simulink model "Simulacion_Trifasico_PID_v8"  (R2024a)
settings: Solver=ode3  StartTime=0  StopTime=tend  FixedStep=0.01  RelTol=1e-3
values from neighbouring files (symbols this model uses):
  ts = 0.1    [Fuzzy_init.m]    (also in MPC_linealizar_v6.m)
libraries: simulink x6, eeStairGenerator x6
settings Model: Creator=Ivan  LastModifiedBy=Ivan
settings DebuggingCC: UnderSpecifiedDimensionMsg=warning
settings ConfigComp: PLC_TargetIDE=tiaportal  PLC_MultiTBSigbuilderTimeRange=off  PLC_FoldFBCallOutputVar=off  PLC_RemoveUnusedSSMethodCallArguments=off  PLC_UseCallOutputArgSyntax=off  PLC_EnableUnsignedAndDoubleTypes=off  PLC_EnableUDTSplitting=off  PLC_MaxFieldsInUDT=500  PLC_InlineEnumCastFunction=off

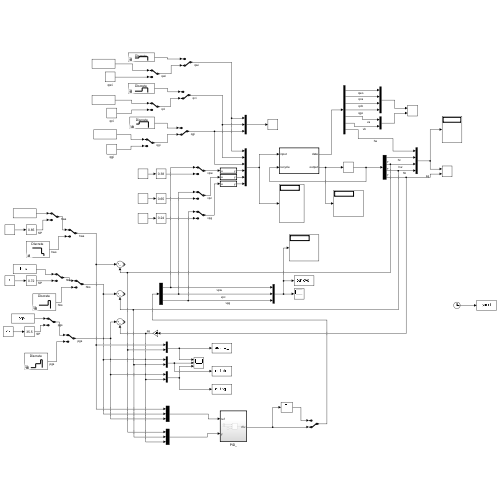
[thumbnail: Simulink's stored preview of the top-level diagram]
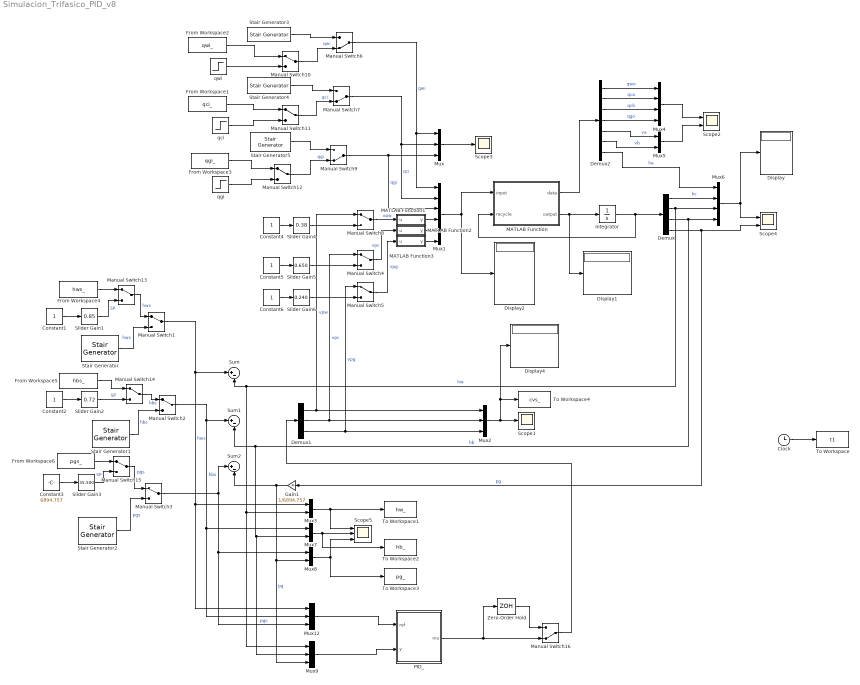
== system Simulacion_Trifasico_PID_v8 ==
  Clock : Clock
  Constant{1..2,4..6} (5 alike) : Constant
  Constant3 : Constant  Value=6894.757
  Demux : Demux
  Demux1 : Demux  Outputs=3
  Demux2 : Demux  Outputs=7
  Display{,1..2,4} (4 alike) : Display
  From Workspace1 : FromWorkspace  VariableName=qci_  SampleTime=ts
  From Workspace2 : FromWorkspace  VariableName=qwi_  SampleTime=ts
  From Workspace3 : FromWorkspace  VariableName=qgi_  SampleTime=ts
  From Workspace4 : FromWorkspace  VariableName=hws_  SampleTime=ts
  From Workspace5 : FromWorkspace  VariableName=hbs_  SampleTime=ts
  From Workspace6 : FromWorkspace  VariableName=pgs_  SampleTime=ts
  Gain1 : Gain  Gain=1/6894.757
  Integrator : Integrator  InitialCondition=[0.4737; 0.80; 0.72; 37*6894.757]  LimitOutput=on  LowerSaturationLimit=0
  MATLAB Function : MATLAB Function  TreatAsAtomicUnit=on
  MATLAB Function1 : MATLAB Function  TreatAsAtomicUnit=on
  MATLAB Function2 : MATLAB Function  TreatAsAtomicUnit=on
  MATLAB Function3 : MATLAB Function  TreatAsAtomicUnit=on
  Manual Switch{1..5,8,10..15} (12 alike) : ManualSwitch
  Manual Switch{6..7,9,16} (4 alike) : ManualSwitch  CurrentSetting=0
  Mux{,2,9,12} (4 alike) : Mux  Inputs=3
  Mux1 : Mux  Inputs=6
  Mux{3,5,7..8} (4 alike) : Mux  Inputs=2
  Mux4 : Mux
  Mux6 : Mux
  PID_ : Subsystem  TreatAsAtomicUnit=on  SystemSampleTime=0.1
  Scope1 : Scope
  Scope2 : Scope  NumInputPorts=2
  Scope3 : Scope
  Scope4 : Scope  NumInputPorts=2
  Scope5 : Scope  NumInputPorts=3
  Slider Gain1 : simulink/Math Operations/Slider Gain  gain=0.85  low=0  high=1
  Slider Gain2 : simulink/Math Operations/Slider Gain  gain=0.72  low=0  high=1
  Slider Gain3 : simulink/Math Operations/Slider Gain  gain=35.500  low=0  high=50
  Slider Gain4 : simulink/Math Operations/Slider Gain  gain=0.38  low=0  high=1
  Slider Gain5 : simulink/Math Operations/Slider Gain  gain=0.650  low=0  high=1
  Slider Gain6 : simulink/Math Operations/Slider Gain  gain=0.240  low=0  high=1
  Stair Generator : eeStairGenerator/Stair Generator  LabelModeActiveChoice=Discrete  TimeInput=[0 2000 2500]  AmplitudeInput=[0.85 0.80 0.78]  SampleTime=0.01  RepeatPattern=off  OutDataTypeStr=double
      settings: LibrarySourceBlock=ee_sl_lib/General Control/Stair Generator
  Stair Generator1 : eeStairGenerator/Stair Generator  LabelModeActiveChoice=Discrete  TimeInput=[0 2250 2750]  AmplitudeInput=[0.72 0.75 0.70]  SampleTime=0.01  RepeatPattern=off  OutDataTypeStr=double
      settings: LibrarySourceBlock=ee_sl_lib/General Control/Stair Generator
  Stair Generator2 : eeStairGenerator/Stair Generator  LabelModeActiveChoice=Discrete  TimeInput="[0 1500 3000  3500]"  AmplitudeInput=[35 40 45 35]  SampleTime=0.01  RepeatPattern=off  OutDataTypeStr=double
      settings: LibrarySourceBlock=ee_sl_lib/General Control/Stair Generator
  Stair Generator3 : eeStairGenerator/Stair Generator  LabelModeActiveChoice=Discrete  TimeInput=[0 1000 3250]  AmplitudeInput=[0.1374 0.1774 0.0474]  SampleTime=0.01  RepeatPattern=off  OutDataTypeStr=double
      settings: LibrarySourceBlock=ee_sl_lib/General Control/Stair Generator
  Stair Generator4 : eeStairGenerator/Stair Generator  LabelModeActiveChoice=Discrete  TimeInput=[0 1750 3100]  AmplitudeInput=[0.0711 0.1815 0.0298]  SampleTime=0.01  RepeatPattern=off  OutDataTypeStr=double
      settings: LibrarySourceBlock=ee_sl_lib/General Control/Stair Generator
  Stair Generator5 : eeStairGenerator/Stair Generator  LabelModeActiveChoice=Discrete  TimeInput=[0 1000 3750]  AmplitudeInput=[0.4906 0.79606 0.006]  SampleTime=0.01  RepeatPattern=off  OutDataTypeStr=double
      settings: LibrarySourceBlock=ee_sl_lib/General Control/Stair Generator
  Sum : Sum  Inputs=|+-
  Sum1 : Sum  Inputs=|+-
  Sum2 : Sum  Inputs=|+-
  To Workspace : ToWorkspace  VariableName=t1  SampleTime=0.1
  To Workspace1 : ToWorkspace  VariableName=hw_  SampleTime=0.1
  To Workspace2 : ToWorkspace  VariableName=hb_  SampleTime=0.1
  To Workspace3 : ToWorkspace  VariableName=pg_  SampleTime=0.1
  To Workspace4 : ToWorkspace  VariableName=cvs_  SampleTime=0.1
  Zero-Order Hold : ZeroOrderHold  SampleTime=-1
  qci : Step  After=.0711  SampleTime=0
  qgi : Step  After=.4906  SampleTime=0
  qwi : Step  After=.1374  SampleTime=0
  wires:
  Mux/1 -> Scope3/1
  Demux2/1 -> Mux4/1  "qwo"
  Demux2/2 -> Mux4/2  "qca"
  Demux2/3 -> Mux4/3  "qcb"
  Demux2/4 -> Mux4/4  "qgo"
  Demux2/5 -> Mux5/1  "va"
  Demux2/6 -> Mux5/2  "vb"
  Mux4/1 -> Scope2/1
  Mux5/1 -> Scope2/2
  Demux2/7 -> Mux6/1  "ha"
  Integrator/1 -> MATLAB Function/2(recycle), Demux/1
  Demux/1 -> Mux6/2  "hc"
  Demux/2 -> Mux9/1, Mux3/2, Sum/2, Mux6/3  "hw"
  Demux/3 -> Mux6/4, Sum1/2, Mux9/2, Mux7/2  "hb"
  Mux6/1 -> Display/1, Scope4/1
  Demux/4 -> Gain1/1, Scope4/2  "pg"
  Mux1/1 -> MATLAB Function/1(input), Display2/1
  MATLAB Function/2(output) -> Display1/1, Integrator/1
  MATLAB Function/1(data) -> Demux2/1
  Mux3/1 -> Scope5/1, To Workspace1/1
  Mux7/1 -> To Workspace2/1, Scope5/2
  Mux8/1 -> To Workspace3/1, Scope5/3
  Constant1/1 -> Slider Gain1/1
  Manual Switch1/1 -> Sum/1, Mux12/1, Mux3/1  "hws"
  Stair Generator/1 -> Manual Switch1/2  "hws"
  Constant2/1 -> Slider Gain2/1
  Manual Switch2/1 -> Sum1/1, Mux12/2, Mux7/1  "hbs"
  Constant3/1 -> Slider Gain3/1
  Manual Switch3/1 -> Sum2/1, Mux8/1, Mux12/3  "pgs"
  Stair Generator1/1 -> Manual Switch2/2  "hbs"
  Stair Generator2/1 -> Manual Switch3/2  "pgs"
  Constant4/1 -> Slider Gain4/1
  Slider Gain4/1 -> Manual Switch8/2
  Slider Gain5/1 -> Manual Switch4/2
  Constant5/1 -> Slider Gain5/1
  Slider Gain6/1 -> Manual Switch5/2
  Constant6/1 -> Slider Gain6/1
  Stair Generator3/1 -> Manual Switch6/1
  Stair Generator4/1 -> Manual Switch7/1
  Stair Generator5/1 -> Manual Switch9/1
  Manual Switch6/1 -> Mux1/1, Mux/1  "qwi"
  Manual Switch7/1 -> Mux/2, Mux1/2  "qci"
  Manual Switch9/1 -> Mux/3, Mux1/3  "qgi"
  Clock/1 -> To Workspace/1
  qwi/1 -> Manual Switch10/2
  Manual Switch10/1 -> Manual Switch6/2  "qwi"
  From Workspace2/1 -> Manual Switch10/1
  qci/1 -> Manual Switch11/2
  Manual Switch11/1 -> Manual Switch7/2  "qci"
  From Workspace1/1 -> Manual Switch11/1
  qgi/1 -> Manual Switch12/2
  Manual Switch12/1 -> Manual Switch9/2  "qgi"
  From Workspace3/1 -> Manual Switch12/1
  Slider Gain1/1 -> Manual Switch13/2  "SP"
  Manual Switch13/1 -> Manual Switch1/1  "hws"
  Slider Gain2/1 -> Manual Switch14/2  "SP"
  Manual Switch14/1 -> Manual Switch2/1  "hbs"
  Manual Switch15/1 -> Manual Switch3/1  "pgs"
  Slider Gain3/1 -> Manual Switch15/2  "SP"
  From Workspace4/1 -> Manual Switch13/1
  From Workspace5/1 -> Manual Switch14/1
  From Workspace6/1 -> Manual Switch15/1
  Manual Switch8/1 -> MATLAB Function1/1(u)  "vpw"
  Manual Switch4/1 -> MATLAB Function2/1(u)  "vpc"
  Manual Switch5/1 -> MATLAB Function3/1(u)  "vpg"
  MATLAB Function1/1(y) -> Mux1/4
  MATLAB Function2/1(y) -> Mux1/5
  MATLAB Function3/1(y) -> Mux1/6
  Gain1/1 -> Mux9/3, Mux8/2, Sum2/2  "pg"
  Mux2/1 -> Display4/1, To Workspace4/1, Scope1/1
  Demux1/3 -> Mux2/3, Manual Switch5/1  "vpg"
  Demux1/1 -> Manual Switch8/1, Mux2/1  "vpw"
  Demux1/2 -> Mux2/2, Manual Switch4/1  "vpc"
  Zero-Order Hold/1 -> Manual Switch16/1
  Manual Switch16/1 -> Demux1/1
  PID_/1(mv) -> Zero-Order Hold/1, Manual Switch16/2
  Mux12/1 -> PID_/1(ref)
  Mux9/1 -> PID_/2(y)

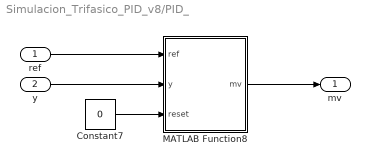
== system Simulacion_Trifasico_PID_v8/PID_ ==
  ref : Inport
  y : Inport  Port=2
  Constant7 : Constant  Value=0
  MATLAB Function8 : MATLAB Function  TreatAsAtomicUnit=on
  mv : Outport
  wires:
  ref/1 -> MATLAB Function8/1(ref)
  MATLAB Function8/1(mv) -> mv/1
  y/1 -> MATLAB Function8/2(y)
  Constant7/1 -> MATLAB Function8/3(reset)

== matlab function Simulacion_Trifasico_PID_v8/MATLAB Function2 ==
  data: u input; y output
function y = fcn(u)

% y = 1-tanh(u);
y = (u);

== matlab function Simulacion_Trifasico_PID_v8/MATLAB Function ==
  data: input input size=6; data output size=7; output output size=4; recycle input size=4
function [data, output] = tpsep_v11(input, recycle)
% Modelo dinamico corregido para NMPC/Simulink.
% Estado: recycle = [hc hw hb pg_Pa]
% Entrada: input = [qwi qci qgi vpw vpc vpg]

% qwi = input(1);
% qci = input(2);
% qgi = input(3);
% vpw = min(max(input(4),0),1);
% vpc = min(max(input(5),0),1);
% vpg = min(max(input(6),0),1);

%% Inputs
qwi = input(1);             % Flujo de entrada agua     [m3/s]
qci = input(2);             % Flujo de entrada crudo    [m3/s]
qgi = input(3);             % Flujo de entrada gas      [m3/s]
vpw = input(4);             % Apertura válvula agua     [-]
vpc = input(5);             % Apertura válvula crudo    [-]
vpg = input(6);             % Apertura válvula gas      [-]

%% DATA (parámetros del separador)
constants = [3.048,...   %1 Diámetro del separador    [m] 10ft
             15.1724,...  %2 Longitud separador        [m] 50ft
             3.1076,...  %3 Longitud colector         [m] 10ft
             1.2192,...  %4 Altura barrera            [m] 4ft   1.2192
             5.15e-4,...  %5 Coef. válvula agua        [m^3/s Pa^0.5]
             101325,...  %6 Presión salida v.agua     [Pa]
             7.15e-4,...  %7 Coef. válvula crudo       [m^3/s Pa^0.5]
             101325,...  %8 Presión salida v.crudo    [Pa]
             80.0,...    %9 Coef. válvula gas         [gpm/psi^0.5]
             101325,...  %10 Presión salida v.gas      [Pa]
             802.525,... %11 Densidad crudo            [kg/m^3]
             0.9134,...  %12 Gravedad esp. crudo       [-]
             997.8,...   %13 Densidad agua             [kg/m^3]
             1.00,...    %14 Gravedad esp. agua        [-]
             28.04,...   %15 Peso molecular gas        [g/mol]
             28.96,...   %16 Peso molecular aire       [g/mol]
             9.81,...    %17 Gravedad                  [m/s^2]
             355.37,...  %18 Temperatura               [K] (180°F)
            ];

%% Constantes
ds   = constants(1);        % Diámetro separador [m]
La   = constants(2);        % Longitud separador [m]
Lb   = constants(3);        % Longitud colector  [m]
hs   = constants(4);        % Altura barrera     [m]
kvw  = constants(5);        % Coef. válvula agua [m^3/s Pa^0.5]
poa  = constants(6);        % P salida v.agua    [Pa]
kvc  = constants(7);        % Coef. válvula crudo[m^3/s Pa^0.5]
pob  = constants(8);        % P salida v.crudo   [Pa]
kvg  = constants(9);        % Coef. válvula gas  [gpm/psi^0.5]
poc  = constants(10);       % P salida v.gas     [Pa]
rhoc = constants(11);       % Densidad crudo     [kg/m^3]
sgc  = constants(12);       % Gravedad esp. crudo[-]
rhow = constants(13);       % Densidad agua      [kg/m^3]
sgw  = constants(14);       % Gravedad esp. agua [-]
mgas = constants(15);       % PM gas             [g/mol]
mair = constants(16);       % PM aire            [g/mol]
g    = constants(17);       % Gravedad           [m/s^2]
T    = constants(18);       % Temperatura        [K]

%% Estado previo (recycle)
hc = recycle(1);            % Nivel crudo A [m]
hw = recycle(2);            % Nivel agua    [m]
hb = recycle(3);            % Nivel crudo B [m]
pg = recycle(4);            % Presión gas   [Pa]

hc = max(min(real(hc),hs-1e-6),1e-6);
hw = max(min(real(hw),hs-1e-6),1e-6);
hb = max(min(real(hb),2.5),1e-6);
pg = max(real(pg),1000);

%% Parámetros calculados
vt = hemivolt(ds,La,Lb);    % Volumen total separador [m^3]
ha = hw + hc;               % Altura total líquido A  [m]

% Flujo de líquido hacia el colector (presa, Perry)
if ha <= hs
    qca = 0;
else
    H = max(ha - hs,0);
    qca = 0.415*max(ds - 0.2*H,0)*(H^1.5)*sqrt(2*g);
    if ~isfinite(qca) || qca < 0
        qca = 0;
    end
end

% Flujo de salida de crudo del colector
if hb <= 0
    qcb = 0;
else
    argcb = (pg + rhoc*g*hb - pob)/sgc;
    if argcb <= 0
        qcb = 0;
    else
        qcb = kvc*vpc*sqrt(argcb);
    end
    if ~isfinite(qcb) || qcb < 0
        qcb = 0;
    end
end

% Flujo de salida de agua de la cámara de separación
argwo = (pg + rhoc*g*hc + rhow*g*hw - poa)/sgw;
if argwo <= 0
    qwo = 0;
else
    qwo = kvw*vpw*sqrt(argwo);
end
if ~isfinite(qwo) || qwo < 0
    qwo = 0;
end

% Flujo de salida de gas (ecuación de válvula/gas)
% Gas: pg y poc estan en Pa; la ecuacion usa psia.
Tf = ((T - 273.15)*(9/5)) + 32; % [°F]
pg_psia  = pg*1.450377e-4 + 14.7;
poc_psia = poc*1.450377e-4 + 14.7;

% Solo hay flujo de salida si pg interna supera la presion de salida.
dp2 = pg_psia^2 - poc_psia^2; % qgnum
qgden = (mgas/mair)*(Tf + 460);

if dp2 <= 0 || qgden <= 0 || vpg <= 0
    qgo = 0;
else
    qgo = 962*kvg*vpg*sqrt(dp2/qgden)*7.86579e-6;
end
if ~isfinite(qgo) || qgo < 0
    qgo = 0;
end

% Volúmenes por sección
ha_vol = min(max(ha,0),ds);
hb_vol = min(max(hb,0),ds);

va = hemivols(ha_vol,La,ds);
vb = hemivols(hb_vol,Lb,ds);

%% Modelo (Ecuaciones diferenciales)
eps_h = 1e-4;
dhc = (qci - qca) / hemihead(max(hc,eps_h), ds, La);
dhw = (qwi - qwo) / hemihead(max(hw,eps_h), ds, La);

if ha <= hs
    dhb = 0;
else
    % evita singularidad en h=0
    dhb = (qca - qcb) / hemihead(max(hb,eps_h), ds, Lb);
end

Vgas = max(vt - va - vb,1e-3);
dpg = pg*(qgi - qgo + qci + qwi - qwo - qcb)/Vgas;

if ~isfinite(dpg)
    dpg = 0;
end

%% Salidas
data   = [qwo; qca; qcb; qgo; va; vb; ha];
output = [dhc; dhw; dhb; dpg];

end

== matlab function Simulacion_Trifasico_PID_v8/MATLAB Function3 ==
  data: u input; y output
function y = fcn(u)

% y = 1-tanh(u);
y = (u);

== matlab function Simulacion_Trifasico_PID_v8/MATLAB Function1 ==
  data: u input; y output
function y = fcn(u)

% y = 1-tanh(u);
y = (u);

== matlab function Simulacion_Trifasico_PID_v8/PID_/MATLAB Function8 ==
  settings: updateMethod=DISCRETE
  data: ref input; y input; mv output; reset input
function mv = PID_Controller(ref, y, reset)
%#codegen
% ==========================================================
% PID DISCRETO TPSEP - v8 (simplificada)
%
%   u(k) = u(k-1) + q0*e(k) + q1*e(k-1) + q2*e(k-2)
%
%   q0 =  Kp*( 1 + Ts/(2*Ti) +   Td/Ts )
%   q1 = -Kp*( 1 - Ts/(2*Ti) + 2*Td/Ts )
%   q2 =  Kp*Td/Ts
%
% La salida u ES la apertura de valvula, saturada en [0.01, 0.99].
% Las tres valvulas son de SALIDA (abrir hace BAJAR la PV), por eso
% el error se toma como e = y - ref (accion inversa).
%
% Entradas: ref = [hw_sp; hb_sp; pg_sp], y = [hw; hb; pg], reset
% Salida:   mv  = [vpw; vpc; vpg]
% ==========================================================

Ts = 0.1;                          % [s] periodo de ejecucion real

% ==========================================================
% SINTONIA   (zeta ~ 0.5  ->  sobrepico ~16%)
% ==========================================================
%          hw       hb       pg
Kp = [  53.93;  14.395;   2.673];    % antes 38.52 y 8.941
Ti = [   7.821;  2.702;   1.050];    % antes 10.95 y 4.350

Td = [   0.00;   0.000;   0.000];

% ==========================================================
% LIMITES Y ARRANQUE
% ==========================================================
mv_min   = 0.01;
mv_max   = 0.99;
rate_max = [0.030; 0.030; 0.030];      % por llamada = 0.30 /s con Ts = 0.1
mv0      = [0.6846; 0.2532; 0.4889];   % aperturas de equilibrio

% ==========================================================
% COEFICIENTES
% ==========================================================
q0 =  Kp .* (1.0 + Ts./(2.0.*Ti) +       Td./Ts);
q1 = -Kp .* (1.0 - Ts./(2.0.*Ti) + 2.0.*Td./Ts);
q2 =  Kp .*  Td ./ Ts;

% ==========================================================
% MEMORIAS
% ==========================================================
persistent e1 e2 u last_mv inicializado

if isempty(inicializado) || reset ~= 0
    e1 = zeros(3,1);
    e2 = zeros(3,1);
    u  = mv0;
    last_mv = mv0;
    inicializado = true;
end

% ==========================================================
% LEY DE CONTROL
% ==========================================================
e = y(:) - ref(:);                      % accion inversa

u = u + q0.*e + q1.*e1 + q2.*e2;

for i = 1:3                             % saturacion con memoria saturada
    if u(i) > mv_max                    % (anti-windup de la forma incremental)
        u(i) = mv_max;
    elseif u(i) < mv_min
        u(i) = mv_min;
    end
end

% ==========================================================
% LIMITADOR DE VELOCIDAD
% ==========================================================
mv = u;
for i = 1:3
    d = u(i) - last_mv(i);
    if d > rate_max(i)
        mv(i) = last_mv(i) + rate_max(i);
    elseif d < -rate_max(i)
        mv(i) = last_mv(i) - rate_max(i);
    end
end

last_mv = mv;
e2 = e1;
e1 = e;

end
